simulink model "ElectricVehicleThermalManagementWithHeatPump"  (R2024b)
settings: Solver=VariableStepAuto  StartTime=0.0  StopTime=3600  RelTol=1e-3  AbsTol=1e-3
PreLoadFcn:
  | init_nmpc
InitFcn:
  | init_nmpc
model workspace: external: MATLAB File ElectricVehicleThermalManagementWithHeatPumpParameters.m (data not in the file)
values from neighbouring files (symbols this model uses):
  battery_C1_LUT = [1913.6 12447 30609 ... (first row only)    [ElectricVehicleThermalManagementWithHeatPumpParameters.m]
  battery_capacity_LUT = [280.081 276.25 276.392]    [ElectricVehicleThermalManagementWithHeatPumpParameters.m]
  battery_cell_cp = 795    [ElectricVehicleThermalManagementWithHeatPumpParameters.m]
  battery_cell_mass = 2.5    [ElectricVehicleThermalManagementWithHeatPumpParameters.m]
  battery_Em_LUT = [3.4966 3.5057 3.5148 ... (first row only)    [ElectricVehicleThermalManagementWithHeatPumpParameters.m]
  battery_N_cells = 20    [ElectricVehicleThermalManagementWithHeatPumpParameters.m]
  battery_Qe_init = 0    [ElectricVehicleThermalManagementWithHeatPumpParameters.m]
  battery_R0_LUT = [0.0117 0.0085 0.009 ... (first row only)    [ElectricVehicleThermalManagementWithHeatPumpParameters.m]
  battery_R1_LUT = [0.0109 0.0029 0.0013 ... (first row only)    [ElectricVehicleThermalManagementWithHeatPumpParameters.m]
  battery_SOC_LUT = [0; 0.1; 0.25; 0.5; 0.75; 0.9; 1]    [ElectricVehicleThermalManagementWithHeatPumpParameters.m]
  battery_T_init = -10    [ElectricVehicleThermalManagementWithHeatPumpParameters.m]
  battery_temperature_LUT = [5 20 40]    [ElectricVehicleThermalManagementWithHeatPumpParameters.m]
  cabin_duct_area = 0.04    [ElectricVehicleThermalManagementWithHeatPumpParameters.m]
  cabin_T_init = -10    [ElectricVehicleThermalManagementWithHeatPumpParameters.m]
  chiller_area_primary = 0.43982297150257105    (= 0.439822971503)    [ElectricVehicleThermalManagementWithHeatPumpParameters.m]
  chiller_N_baffles = 3    [ElectricVehicleThermalManagementWithHeatPumpParameters.m]
  chiller_N_tubes = 100    [ElectricVehicleThermalManagementWithHeatPumpParameters.m]
  chiller_tube_D = 0.0035    [ElectricVehicleThermalManagementWithHeatPumpParameters.m]
  chiller_tube_L = 0.4    [ElectricVehicleThermalManagementWithHeatPumpParameters.m]
  chiller_wall_conductivity = 240    [ElectricVehicleThermalManagementWithHeatPumpParameters.m]
  chiller_wall_thickness = 0.0001    [ElectricVehicleThermalManagementWithHeatPumpParameters.m]
  cond_evap_air_area_flow = 0.3906    [ElectricVehicleThermalManagementWithHeatPumpParameters.m]
  cond_evap_air_area_primary = 1.4834999999999998    (= 1.4835)    [ElectricVehicleThermalManagementWithHeatPumpParameters.m]
  cond_evap_W = 0.015    [ElectricVehicleThermalManagementWithHeatPumpParameters.m]
  cond_evap_wall_conductivity = 240    [ElectricVehicleThermalManagementWithHeatPumpParameters.m]
  cond_evap_wall_thickness = 0.0001    [ElectricVehicleThermalManagementWithHeatPumpParameters.m]
  coolant_channel_D = 0.0092    [ElectricVehicleThermalManagementWithHeatPumpParameters.m]
  coolant_pipe_D = 0.019    [ElectricVehicleThermalManagementWithHeatPumpParameters.m]
  coolant_T_init = -10    [ElectricVehicleThermalManagementWithHeatPumpParameters.m]
  coolant_tank_area = 0.0121    [ElectricVehicleThermalManagementWithHeatPumpParameters.m]
  coolant_tank_volume = 1.25    [ElectricVehicleThermalManagementWithHeatPumpParameters.m]
  coolant_valve_D_ratio_max = 0.95    [ElectricVehicleThermalManagementWithHeatPumpParameters.m]
  coolant_valve_D_ratio_min = 0.001    [ElectricVehicleThermalManagementWithHeatPumpParameters.m]
  coolant_valve_displacement = 0.0063    [ElectricVehicleThermalManagementWithHeatPumpParameters.m]
  coolant_valve_S_max = 0.0053    [ElectricVehicleThermalManagementWithHeatPumpParameters.m]
  evaporator_air_area_flow = 0.12    [ElectricVehicleThermalManagementWithHeatPumpParameters.m]
  evaporator_air_area_primary = 0.4323    [ElectricVehicleThermalManagementWithHeatPumpParameters.m]
  evaporator_W = 0.015    [ElectricVehicleThermalManagementWithHeatPumpParameters.m]
  evaporator_wall_conductivity = 240    [ElectricVehicleThermalManagementWithHeatPumpParameters.m]
  evaporator_wall_thickness = 0.0001    [ElectricVehicleThermalManagementWithHeatPumpParameters.m]
  expansion_valve_D_ratio_max = 0.9    [ElectricVehicleThermalManagementWithHeatPumpParameters.m]
  hex_area_primary = 0.070371675440411369    (= 0.0703716754404)    [ElectricVehicleThermalManagementWithHeatPumpParameters.m]
  hex_N_tubes = 64    [ElectricVehicleThermalManagementWithHeatPumpParameters.m]
  hex_tube_D = 0.0035    [ElectricVehicleThermalManagementWithHeatPumpParameters.m]
  hex_wall_conductivity = 240    [ElectricVehicleThermalManagementWithHeatPumpParameters.m]
  hex_wall_thickness = 0.0001    [ElectricVehicleThermalManagementWithHeatPumpParameters.m]
  inner_cond_air_area_flow = 0.1953    [ElectricVehicleThermalManagementWithHeatPumpParameters.m]
  inner_cond_air_area_primary = 0.99520000000000008    (= 0.9952)    [ElectricVehicleThermalManagementWithHeatPumpParameters.m]
  inner_cond_W = 0.02    [ElectricVehicleThermalManagementWithHeatPumpParameters.m]
  inner_cond_wall_conductivity = 240    [ElectricVehicleThermalManagementWithHeatPumpParameters.m]
  inner_cond_wall_thickness = 0.0001    [ElectricVehicleThermalManagementWithHeatPumpParameters.m]
  pump_speed_max = 1000    [ElectricVehicleThermalManagementWithHeatPumpParameters.m]
  radiator_air_area_flow = 0.097499999999999989    (= 0.0975)    [ElectricVehicleThermalManagementWithHeatPumpParameters.m]
  radiator_air_area_primary = 0.43687499999999996    (= 0.436875)    [ElectricVehicleThermalManagementWithHeatPumpParameters.m]
  radiator_W = 0.015    [ElectricVehicleThermalManagementWithHeatPumpParameters.m]
  radiator_wall_conductivity = 240    [ElectricVehicleThermalManagementWithHeatPumpParameters.m]
  radiator_wall_thickness = 0.0001    [ElectricVehicleThermalManagementWithHeatPumpParameters.m]
  refrigerant_p_init = 0.2    [ElectricVehicleThermalManagementWithHeatPumpParameters.m]
  refrigerant_pipe_D = 0.01    [ElectricVehicleThermalManagementWithHeatPumpParameters.m]
  refrigerant_valve_D_ratio_max = 0.95    [ElectricVehicleThermalManagementWithHeatPumpParameters.m]
  refrigerant_valve_displacement = 0.005    [ElectricVehicleThermalManagementWithHeatPumpParameters.m]
libraries: fl_lib x227, nesl_utility x162, SimscapeFluids_lib x30, LiBatteryElements_lib x16, slpidlib x3, SignalEditorBlockLib x1
(part 2 of 13)

== system ElectricVehicleThermalManagementWithHeatPump/Battery Pump ==
  Battery Coolant Tank : SimscapeFluids_lib/Thermal Liquid/Tanks & Accumulators/Tank (G-TL)  num_inlet=2  volume_total=coolant_tank_volume l  volume_spec=1  tank_area=coolant_tank_area m^2  level_TLU=[0, 3, 5] m  volume_TLU=[0, 4, 6] m^3  inlet_areas_A1B1=[.01, .01] m^2  inlet_height_A2=0.1 m  inlet_area_A2=0.01 m^2  inlet_heights_A2B2=[0, 0] m  inlet_areas_A2B2=[1 1] * pi * coolant_pipe_D^2 / 4 m^2  inlet_heights_A2B2C2=[.1, .05, 0] m  inlet_areas_A2B2C2=[.01, .01, .01] m^2  inlet_heights_A2B2C2D2=0.1 * ones(1, 4) m  inlet_areas_A2B2C2D2=0.01 * ones(1, 4) m^2  inlet_heights_A2B2C2D2E2=0.1 * ones(1, 5) m  inlet_areas_A2B2C2D2E2=0.01 * ones(1, 5) m^2  inlet_heights_A2B2C2D2E2F2=0.1 * ones(1, 6) m  inlet_areas_A2B2C2D2E2F2=0.01 * ones(1, 6) m^2  capacity_check=0  max_liquid_capacity=coolant_tank_volume l  g=0 m/s^2  level_specify=on  level_priority=None  level=5 m  level_nominal_specify=off  level_nominal_value=1  level_nominal_unit=m  volume_liquid_specify=on  volume_liquid_priority=High  volume_liquid=0.25 * coolant_tank_volume l  volume_liquid_nominal_specify=off  volume_liquid_nominal_value=1  volume_liquid_nominal_unit=m^3  mass_liquid_specify=off  mass_liquid_priority=None  mass_liquid=5e+3 kg  mass_liquid_nominal_specify=off  mass_liquid_nominal_value=1  mass_liquid_nominal_unit=kg  T_liquid_specify=on  T_liquid_priority=High  T_liquid=coolant_T_init degC  T_liquid_nominal_specify=off  T_liquid_nominal_value=1  T_liquid_nominal_unit=K  p_gas_specify=on  p_gas_priority=High  p_gas=coolant_p_init MPa  p_gas_nominal_specify=off  p_gas_nominal_value=1  p_gas_nominal_unit=MPa  T_gas_specify=on  T_gas_priority=High  T_gas=coolant_T_init degC  T_gas_nominal_specify=off  T_gas_nominal_value=1  T_gas_nominal_unit=K  rho_gas_specify=off  rho_gas_priority=None  rho_gas=1.2 kg/m^3  rho_gas_nominal_specify=off  rho_gas_nominal_value=1  rho_gas_nominal_unit=kg/m^3
      settings: InternalSimscapePortConfiguration="{\"Bottom\":[],\"Left\":[{\"id\":\"A1\",\"label\":\"A1\",\"type\":\"foundation.gas.gas\"},{\"id\":\"B1\",\"label\":\"B1\",\"type\":\"foundation.gas.gas\"},{\"id\":\"A2\",\"label\":\"A2\",\"type\":\"foundation.thermal_liquid.thermal_liquid\"},{\"id\":\"B2\",\"label\":\"B2\",\"type\":\"foundation.thermal_liquid.thermal_liquid\"}],\"Right\":[{\"id\":\"H1\",\"label\":\"H1\",\"type\":\"foundation.thermal.thermal\"},{\"id\":\"H2\",\"label\":\"H2\",\"type\":\"foundation.thermal.thermal\"}],\"Top\":[{\"id\":\"V_out\",\"label\":\"V\",\"type\":\"output\"},{\"id\":\"L_out\",\"label\":\"L\",\"type\":\"output\"}]}"
  Battery Pump : SimscapeFluids_lib/Thermal Liquid/Pumps & Motors/Fixed-Displacement Pump (TL)  loss_spec=1  displacement=pump_displacement l/rev  omega_nominal=0.5 * pump_speed_max rpm  p_nominal=0.1 MPa  mu_nominal=0.9 cP  vol_eff_nominal=0.92  mech_eff_nominal=0.88  no_load_torque=0.03 N*m  p_diff_eff_TLU=[.1, 1, 2] MPa  omega_eff_TLU=[25, 50, 100, 200, 300, 400] rad/s  vol_eff_TLU=[.816, .908, .954, .977, .981, .984; .325, .663, .831, .916, .925, .946; .137, .568, .78, .892, .893, .91]  mech_eff_TLU=[.996, .996, .996, .996, .996, .996; .988, .989, .989, .989, .989, .99; .981, .981, .982, .982, .983, .984]  p_diff_loss_TLU=[.1, 1, 2] MPa  omega_loss_TLU=[25, 50, 100, 200, 300, 400] rad/s  vol_loss_TLU=[.023, .023, .023, .023, .0285, .032; .0844, .0842, .0845, .084, .1125, .108; .1079, .108, .11, .108, .1605, .18] * 1e-3 m^3/s  mech_loss_TLU=[.002, .002, .002, .002, .002, .002; .0607, .0556, .0556, .0556, .0556, .0505; .1937, .1937, .1833, .1833, .1729, .1626] N*m  vol_eff_min=1e-3  vol_eff_max=1  mech_eff_min=1e-3  mech_eff_max=1  pressure_threshold=1e-3 MPa  omega_threshold=10 rad/s  area=pi * coolant_pipe_D^2 / 4 m^2  supplied_range_check=0  pump_mode_check=simscape.enum.assert.action.none  pressure_check=simscape.enum.assert.action.none  p_min_valid=0.101325 MPa
  Cap (G) : fl_lib/Gas/Elements/Cap (G)  p_specify=off  p_priority=None  p=0.101325 MPa  p_nominal_specify=off  p_nominal_value=1  p_nominal_unit=MPa  T_specify=off  T_priority=None  T=293.15 K  T_nominal_specify=off  T_nominal_value=1  T_nominal_unit=K
  Cap (G)1 : fl_lib/Gas/Elements/Cap (G)  p_specify=off  p_priority=None  p=0.101325 MPa  p_nominal_specify=off  p_nominal_value=1  p_nominal_unit=MPa  T_specify=off  T_priority=None  T=293.15 K  T_nominal_specify=off  T_nominal_value=1  T_nominal_unit=K
  Flow Rate Sensor (TL) : fl_lib/Thermal Liquid/Sensors/Flow Rate Sensor (TL)  mass_flow_measure=true  volumetric_flow_measure=false  energy_flow_measure=true
      settings: InternalSimscapePortConfiguration="{\"Bottom\":[{\"id\":\"PHI\",\"label\":\"φ\",\"type\":\"output\"}],\"Left\":[{\"id\":\"A\",\"label\":\"A\",\"type\":\"foundation.thermal_liquid.thermal_liquid\"}],\"Right\":[{\"id\":\"B\",\"label\":\"B\",\"type\":\"foundation.thermal_liquid.thermal_liquid\"},{\"id\":\"M\",\"label\":\"M\",\"type\":\"output\"}],\"Top\":[]}"
  Flow Rate Sensor (TL)1 : fl_lib/Thermal Liquid/Sensors/Flow Rate Sensor (TL)  mass_flow_measure=true  volumetric_flow_measure=false  energy_flow_measure=true
      settings: InternalSimscapePortConfiguration="{\"Bottom\":[{\"id\":\"PHI\",\"label\":\"φ\",\"type\":\"output\"}],\"Left\":[{\"id\":\"A\",\"label\":\"A\",\"type\":\"foundation.thermal_liquid.thermal_liquid\"}],\"Right\":[{\"id\":\"B\",\"label\":\"B\",\"type\":\"foundation.thermal_liquid.thermal_liquid\"},{\"id\":\"M\",\"label\":\"M\",\"type\":\"output\"}],\"Top\":[]}"
  Heat Transfer : Subsystem
  Ideal Angular Velocity Source : fl_lib/Mechanical/Mechanical Sources/Ideal Angular Velocity Source
  Max Speed [rpm] : Gain  Gain=4000
  Mechanical Rotational Reference : fl_lib/Mechanical/Rotational Elements/Mechanical Rotational Reference
  PS-Simulink Converter : nesl_utility/PS-Simulink Converter  PhysicalDomain=network_engine_domain  SubClassName=ps_output  LeftPortType=input  RightPortType=output  PseudoPeriodic=off  Frequencies=[]  VectorFormat=inherit  Unit=kg/s  AffineConversion=off
  PS-Simulink Converter1 : nesl_utility/PS-Simulink Converter  PhysicalDomain=network_engine_domain  SubClassName=ps_output  LeftPortType=input  RightPortType=output  PseudoPeriodic=off  Frequencies=[]  VectorFormat=inherit  Unit=inherit  AffineConversion=off
  Scope : Scope
  Scope1 : Scope
  Simulink-PS Converter : nesl_utility/Simulink-PS Converter  PhysicalDomain=network_engine_domain  SubClassName=ps_input  LeftPortType=input  RightPortType=output  PseudoPeriodic=off  Frequencies=[]  NoiseDistribution=none  NoiseParameters=[]  Unit=rpm  AffineConversion=off  FilteringAndDerivatives=provide  SimscapeFilterOrder=1  InputFilterTimeConstant=0.001  UdotUserProvided=0
  Switch : Switch  Criteria=u2 > Threshold  SaturateOnIntegerOverflow=off  InputSameDT=off
  Transfer Fcn : TransferFcn  Denominator=[5 1]
  Transfer Fcn1 : TransferFcn  Denominator=[5 1]
  A : PMIOPort  Side=Left
  B : PMIOPort  Port=2  Side=Right
  wires:
  Transfer Fcn/1 -> Max Speed [rpm]/1
  [cmd_battery_pump] -> Transfer Fcn/1
  PS-Simulink Converter/1 -> Scope/1
  PS-Simulink Converter1/1 -> Scope1/1
  [batPumpNrpm] -> Transfer Fcn1/1
  [MPCController] -> Switch/2
  Max Speed [rpm]/1 -> Switch/3
  Switch/1 -> Simulink-PS Converter/1
  Transfer Fcn1/1 -> Switch/1
  connections:
  Mechanical Rotational Reference/LConn1 -- Ideal Angular Velocity Source/RConn2 -- Battery Pump/RConn2
  Simulink-PS Converter/RConn1 -- Ideal Angular Velocity Source/RConn1
  Ideal Angular Velocity Source/LConn1 -- Battery Pump/RConn1
  A/RConn1 -- Battery Coolant Tank/LConn3 -- Flow Rate Sensor (TL)/LConn1
  Cap (G)1/LConn1 -- Battery Coolant Tank/LConn2
  Heat Transfer/RConn2 -- Battery Coolant Tank/RConn2
  Cap (G)/LConn1 -- Battery Coolant Tank/LConn1
  Battery Pump/LConn1 -- Battery Coolant Tank/LConn4
  Heat Transfer/RConn1 -- Battery Coolant Tank/RConn1
  Flow Rate Sensor (TL)/RConn2 -- PS-Simulink Converter/LConn1
  Flow Rate Sensor (TL)1/RConn1 -- Battery Pump/LConn2
  Flow Rate Sensor (TL)1/LConn1 -- B/RConn1
  PS-Simulink Converter1/LConn1 -- Flow Rate Sensor (TL)1/RConn2

== system ElectricVehicleThermalManagementWithHeatPump/Blend Door ==
  Blend Door : Subsystem  Tag=PublishSubsystem  mask{min_area=1e-8 * cabin_duct_area, max_area=0.9 * cabin_duct_area, port_area=cabin_duct_area, Cd=0.8, tau=1}
      mask prompts: min_area "Min restriction area (m^2)"; max_area "Max restriction area (m^2)"; port_area "Cross-sectional area at ports A, B, and C (m^2)"; Cd "Discharge coefficient"; tau "Opening time constant (s)"
      settings: PortSchema="{\"entries\":[{\"content\":{\"sides\":[{\"content\":{\"connectorIds\":[\"LConn1\"]},\"type\":\"ConnectorPlacement.EquallySpacedRectSide\",\"uuid\":\"701091b4-901c-43e1-a8a1-50bf4fd327d1\"},{\"content\":{\"connectorIds\":[\"RConn1\"],\"side\":\"RIGHT\"},\"type\":\"ConnectorPlacement.EquallySpacedRectSide\",\"uuid\":\"6ee33cdd-bbd1-4683-8a8c-22edb39550e2\"},{\"content\":{\"side\":\"TOP\"},\"type\":\"ConnectorPlacement.EquallySpacedRectSide\",\"uuid\":\"c0b8be11-b43c-4098-95a0-d44066221ea6\"},{\"content\":{\"connectorIds\":[\"RConn2\"],\"side\":\"BOTTOM\"},\"type\":\"ConnectorPlacement.EquallySpacedRectSide\",\"uuid\":\"1c585638-1e64-4636-940b-c407bc21f999\"}]},\"type\":\"ConnectorPlacement.EquallySpacedConnector\",\"uuid\":\"9280612b-569a-4615-9ade-e87314c5223e\"}],\"packageUris\":[\"http://schema.mathworks.com/mf0/Connector/R2020b\"],\"version\":\"1.0\"}"
  A : PMIOPort  Side=Left
  B : PMIOPort  Port=2  Side=Right
  C : PMIOPort  Port=3  Side=Right
  connections:
  Blend Door/LConn1 -- A/RConn1
  B/RConn1 -- Blend Door/RConn1
  C/RConn1 -- Blend Door/RConn2

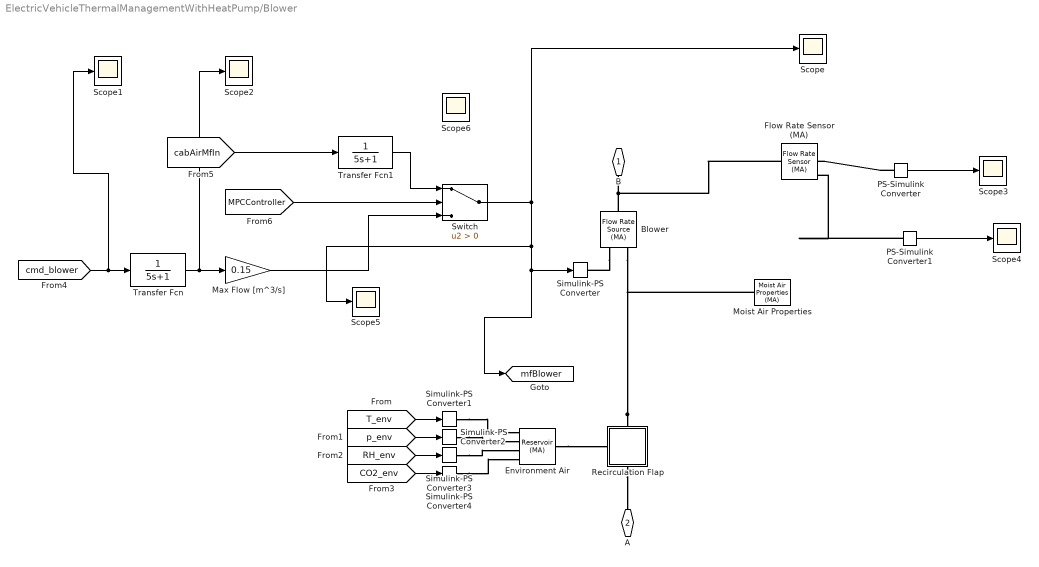
== system ElectricVehicleThermalManagementWithHeatPump/Blower ==
  Blower : fl_lib/Moist Air/Sources/Flow Rate Source (MA)  source_type=foundation.enum.constant_controlled.controlled  flow_type=foundation.enum.mass_volumetric_flow.volumetric  mass_flow=0 kg/s  volumetric_flow=0 m^3/s  volumetric_flow_conditions=foundation.enum.volumetric_flow_conditions.actual  p_std=0.101325 MPa  T_std=20 degC  RH_std=0.65  power_spec=foundation.enum.power_spec.isentropic  area_A=cabin_duct_area m^2  area_B=cabin_duct_area m^2
      settings: InternalSimscapePortConfiguration="{\"Bottom\":[],\"Left\":[{\"id\":\"A\",\"label\":\"A\",\"type\":\"foundation.moist_air.moist_air\"},{\"id\":\"V\",\"label\":\"V\",\"type\":\"input\"}],\"Right\":[{\"id\":\"B\",\"label\":\"B\",\"type\":\"foundation.moist_air.moist_air\"}],\"Top\":[]}"
  Environment Air : fl_lib/Moist Air/Elements/Reservoir (MA)  pressure_input=true  pressure_spec=foundation.enum.pressure_spec.atmospheric  reservoir_pressure=0.101325 MPa  temperature_input=true  temperature_spec=foundation.enum.temperature_spec.atmospheric  reservoir_temperature=293.15 K  humidity_input=true  humidity_spec=foundation.enum.HumiditySpec.RelativeHumidity  reservoir_RH=0.5  reservoir_x_w=0.01  reservoir_y_w=0.01  reservoir_HR=0.01  reservoir_Tw=287 K  trace_gas_input=true  trace_gas_spec=foundation.enum.trace_gas_spec.mole_fraction  reservoir_x_g=0.001  reservoir_y_g=0.001  water_droplets_input=false  reservoir_r_d=0  RH_ws=1  area_A=cabin_duct_area m^2  input_error_spec=foundation.enum.input_range_error.warn
      settings: InternalSimscapePortConfiguration="{\"Bottom\":[],\"Left\":[{\"id\":\"A\",\"label\":\"A\",\"type\":\"foundation.moist_air.moist_air\"}],\"Right\":[{\"id\":\"T\",\"label\":\"T\",\"type\":\"input\"},{\"id\":\"P\",\"label\":\"P\",\"type\":\"input\"},{\"id\":\"W\",\"label\":\"W\",\"type\":\"input\"},{\"id\":\"G\",\"label\":\"G\",\"type\":\"input\"}],\"Top\":[]}"
  Flow Rate Sensor (MA) : fl_lib/Moist Air/Sensors/Flow Rate Sensor (MA)  mass_flow_measure=true  volumetric_flow_measure=false  volumetric_flow_conditions=foundation.enum.volumetric_flow_conditions.actual  p_std=0.101325 MPa  T_std=20 degC  RH_std=0.65  energy_flow_measure=true  vapor_flow_measure=false  gas_flow_measure=false  droplets_flow_measure=false
      settings: InternalSimscapePortConfiguration="{\"Bottom\":[{\"id\":\"PHI\",\"label\":\"φ\",\"type\":\"output\"}],\"Left\":[{\"id\":\"A\",\"label\":\"A\",\"type\":\"foundation.moist_air.moist_air\"}],\"Right\":[{\"id\":\"B\",\"label\":\"B\",\"type\":\"foundation.moist_air.moist_air\"},{\"id\":\"M\",\"label\":\"M\",\"type\":\"output\"}],\"Top\":[]}"
  Max Flow [m^3/s] : Gain  Gain=0.15
  Moist Air Properties : fl_lib/Moist Air/Utilities/Moist Air Properties (MA)  R_a=287.047 J/(K*kg)  T_TLU=[-56.55, -50 : 10 : -10, -5 : 1 : 5, 10 : 10 : 350]' degC  h_a_TLU=[342.414066793634; 349.003411914139; 359.061417476782; 369.117728274935; 379.173188407993; 389.228602960013; 394.256538873206; 395.262156814682; 396.26778682262; 397.27342967397; 398.279086145689; 399.284757014822; 400.290443058569; 401.296145054364; 402.301863779931; 403.307600013352; 404.313354533128; 409.342428711098; 419.402397945314; 429.465451846544; 439.532387826623; 449.604014793745; 459.68115297076; 469.764632657687; 479.855292205971; 489.953975419749; 500.06152856014; 510.178797098051; 520.306622336267; 530.445838000969; 540.597266885076; 550.761717610289; 560.939981561004; 571.132830031086; 581.341011613777; 591.565249855533; 601.806241186423; 612.064653132654; 622.341122810862; 632.636255698901; 642.95062467384; 653.284769304793; 663.639195385783; 674.014374692179; 684.410744943084; 694.828709951456; 705.268639943519; 715.730872029167; 726.215710805484; 736.723429076127; 747.254268670154; 757.808441344776] kJ/kg  mu_a_TLU=[14.2568884161326; 14.6140128551699; 15.151727785151; 15.6806860927178; 16.201235181264; 16.7137043838401; 16.9670072430524; 17.017438132541; 17.0677931537044; 17.1180726001803; 17.1682767640582; 17.2184059358881; 17.2684604046898; 17.318440457962; 17.3683463816913; 17.4181784603614; 17.467936976962; 17.7156359301048; 18.2056752419787; 18.6887904184394; 19.1652345249932; 19.6352479488881; 20.099059157425; 20.5568854116507; 21.008933436444; 21.4554000485251; 21.8964727442509; 22.3323302492491; 22.7631430320408; 23.1890737838183; 23.6102778665211; 24.0269037312887; 24.4390933092858; 24.8469823767971; 25.2507008963847; 25.6503733357905; 26.0461189661617; 26.438052141067; 26.8262825576728; 27.210915501349; 27.5920520748824; 27.969789413389; 28.3442208859359; 28.7154362848061; 29.0835220032714; 29.4485612026716; 29.8106339695395; 30.169817463453; 30.5261860562487; 30.8798114631771; 31.2307628665438; 31.5791070323335] s*uPa  k_a_TLU=[19.8808491891482; 20.4162457047568; 21.2248745869044; 22.0232455041378; 22.8117316528767; 23.59069155438; 23.9767077285082; 24.0536401764626; 24.130482853517; 24.2072360894785; 24.2839002127411; 24.3604755502875; 24.4369624276914; 24.5133611691197; 24.5896720973349; 24.6658955336975; 24.7420317981691; 25.1214166432482; 25.8738284673185; 26.6180151791963; 27.3542675863918; 28.0828636150405; 28.8040688184917; 29.5181369069754; 30.2253102842368; 30.9258205811167; 31.6198891790667; 32.307727718801; 32.989538590917; 33.6655154065126; 34.3358434467079; 35.0007000906151; 35.6602552217624; 36.314671613305; 36.9641052925838; 37.6087058857479; 38.2486169432557; 38.8839762471259; 39.5149161008418; 40.1415636028127; 40.7640409042923; 41.3824654526272; 41.9969502206863; 42.6076039232795; 43.2145312213471; 43.8178329146528; 44.4176061236819; 45.0139444614019; 45.6069381955058; 46.1966744017242; 46.7832371087507; 47.3667074352967] mW/(K*m)  p_min=1 kPa  p_max=inf MPa  T_min=-56.55 degC  T_max=350 degC  properties_range_check=simscape.enum.assert.action.error  p_atm=0.101325 MPa  T_atm=20 degC  enable_droplets=false  R_w=461.523 J/(K*kg)  p_ws_TLU=[1.71168953425982e-06; 3.93770601979424e-06; 1.28411717710344e-05; 3.80051394873809e-05; .00010323902900209; .000259873810798063; .000401741022116384; .000437454836117844; .000476040820618202; .000517704666185737; .000562664883741207; .000611212677444345; .000657085634113763; .000705985593917791; .00075808051438111; .000813548355379396; .000872575113841924; .00122819910164487; .00233931836947519; .00424697076171126; .00738493802968097; .012351945812707; .0199464343236764; .0312009300307261; .0474144740241604; .0701817658485933; .101417996663294; .143378712947169; .198674420476403; .270279976781692; .361539099388177; .476164537971214; .618234621423587; .792187006980199; 1.00281053608169; 1.25523615516845; 1.55492790046272; 1.90767499353199; 2.31958617020155; 2.79708749692822; 3.34692514426746; 3.97617493064794; 4.69226099229504; 5.50298678300951; 6.41658290952841; 7.44177834442093; 8.58790494083256; 9.86505121117553; 11.284292927457; 12.8580516000122; 14.6006773719404; 16.5294151389953] MPa  h_w_vap_TLU=[2836.88241275372; 2837.81392500514; 2838.63937175807; 2838.7309929628; 2838.06905313927; 2836.62597341095; 2835.60023952573; 2835.37006381376; 2835.13143158077; 2834.88429145066; 2834.62859062897; 2500.93420564316; 2498.55452890293; 2496.17317793437; 2493.7941260618; 2491.41713708944; 2489.04199020767; 2477.18706302224; 2453.51925941961; 2429.81122987564; 2405.97728678685; 2381.94712654051; 2357.65452030374; 2333.03120800924; 2308.00352809267; 2282.49062771796; 2256.40372152657; 2229.64615315163; 2202.11407337172; 2173.6974807639; 2144.28128268553; 2113.74600964951; 2081.9678834089; 2048.81807129851; 2014.16109962579; 1977.85249331179; 1939.73572816654; 1899.63852389863; 1857.36838273035; 1812.70710332357; 1765.4037880462; 1715.16561416478; 1661.64526339623; 1604.4232249434; 1542.98206457018; 1476.66790089115; 1404.63083498414; 1325.72875296442; 1238.36212284382; 1140.16281350074; 1027.31658328826; 892.746804215825] kJ/kg  h_w_TLU=[2396.53078650168; 2408.65722023252; 2427.16766028467; 2445.66624034104; 2464.1379798878; 2482.5594701893; 2491.7412703989; 2493.57467660537; 2495.40699233755; 2497.23816944599; 2499.06815833272; 2500.89261781717; 2502.73123919979; 2504.56496564907; 2506.39800457704; 2508.23033644628; 2510.06194120626; 2519.20831890725; 2537.43340437276; 2555.54520329515; 2573.51032237465; 2591.28888786817; 2608.83487221908; 2626.09640083333; 2643.01588134754; 2659.53001419864; 2675.5827869577; 2696.18462565746; 2716.49989554204; 2736.6235211014; 2756.61216047677; 2776.50561774616; 2796.33378923373; 2816.11979584021; 2835.88181424959; 2855.6343057571; 2875.38889328914; 2895.15500578618; 2914.94035966265; 2934.75132291939; 2954.59319332093; 2974.47041287496; 2994.38673461102; 3014.34535330297; 3034.34900869544; 3054.40006758361; 3074.50058949656; 3094.65237956705; 3114.85703131193; 3135.11596141057; 3155.43043809331; 3175.80160439414] kJ/kg  mu_w_TLU=[6.9886414857741; 7.21462000349698; 7.55962537406626; 7.90463074463554; 8.24963611520482; 8.5946414857741; 8.76714417105874; 8.80164470811567; 8.8361452451726; 8.87064578222952; 8.90514631928645; 8.93964685634338; 8.97414739340031; 9.00294911497154; 9.0318980288863; 9.06099135942002; 9.09022638806001; 9.23843559844524; 9.5440595677542; 9.86015858692705; 10.1848429274122; 10.5164578096049; 10.8535319382781; 11.1947482575333; 11.5389294976352; 11.8850331780701; 12.2322493177351; 12.6188533568459; 13.0082793358938; 13.4003380262893; 13.7948421428098; 14.1916095618232; 14.590464747099; 14.9912394314964; 15.3937729006119; 15.7979120385447; 16.203511226482; 16.610432150303; 17.0185435533718; 17.4277209582061; 17.8378463726577; 18.2488079909412; 18.6604998963166; 19.0728217698535; 19.485678608085; 19.8989804512625; 20.3126421231677; 20.7265829829225; 21.1407266888906; 21.5550009745266; 21.969337435876; 22.3836713303269] s*uPa  k_w_TLU=[12.4916816538045; 12.9847788176262; 13.737598915064; 14.4904190125018; 15.2432391099396; 15.9960592073774; 16.3724692560963; 16.4477512658401; 16.5230332755839; 16.5983152853277; 16.6735972950715; 16.7488793048152; 16.824161314559; 16.8886088206517; 16.9532779906513; 17.0181691764255; 17.083282769915; 17.4122036181723; 18.0870861656185; 18.7855813517187; 19.5093466408385; 20.2607864040347; 21.0430876297671; 21.8602068151121; 22.7168164077153; 23.6182141540994; 24.5698636875305; 25.4024944426483; 26.2458938647479; 27.1009155051916; 27.968142896353; 28.8479507975112; 29.7405485790829; 30.646029672269; 31.5643932662527; 32.4955693285114; 33.4394360046859; 34.3958329885356; 35.3645718140131; 36.3454437886179; 37.3382261129791; 38.3426866012072; 39.3585873185985; 40.3856873794121; 41.4237450915028; 42.4725195920623; 43.5317720862424; 44.6012667755489; 45.6807715437344; 46.7700584531355; 47.8689040929333; 48.9770898119082] mW/(K*m)  D_w=25 mm^2/s  trace_gas_model=foundation.enum.trace_gas_model.track_fraction  R_g=188.923 J/(K*kg)  h_g_TLU=[439.555216276024; 444.670268214299; 452.538618857965; 460.487124266174; 468.522588773143; 476.64941595933; 480.747985385885; 481.570543185868; 482.394052396612; 483.218514286302; 484.043930026094; 484.87030069324; 485.697627274149; 486.525910667382; 487.355151686572; 488.185351063277; 489.016509449741; 493.186704132078; 501.599194941473; 510.107689945701; 518.711611059603; 527.410026767716; 536.20176474847; 545.085474167968; 554.059675464379; 563.122805439004; 572.273250917104; 581.509372969931; 590.829525041787; 600.232066635428; 609.715373504524; 619.277845094572; 628.91790983254; 638.634028741375; 648.424697754692; 658.288449028076; 668.22385148184; 678.229510761734; 688.30406876583; 698.446202855373; 708.654624842952; 718.928079831753; 729.265344963773; 739.665228122078; 750.126566621791; 760.648225916092; 771.229098336723; 781.86810188302; 792.564179069104; 803.316295835373; 814.123440527678; 824.984622945405] kJ/kg  mu_g_TLU=[10.9386626034033; 11.2618160869372; 11.7542862475187; 12.2454955799777; 12.7352208796158; 13.2232325321233; 13.4665248390743; 13.5151226761166; 13.5636997995993; 13.6122559954699; 13.6607910510226; 13.709304754931; 13.757796897279; 13.8062672695897; 13.8547156648526; 13.9031418775498; 13.9515457036801; 14.1932220047332; 14.6747828595747; 15.153802214283; 15.6301123398299; 16.1035631756244; 16.574022106427; 17.0413733976215; 17.5055174102327; 17.9663696812767; 18.4238599299346; 18.8779310322956; 19.3285379947687; 19.7756469471288; 20.2192341695255; 20.6592851629269; 21.0957937689132; 21.5287613421341; 21.9581959768344; 22.3841117874779; 22.8065282425078; 23.2254695495877; 23.6409640901974; 24.0530439011453; 24.4617442003854; 24.8671029544344; 25.269160484669; 25.6679591098169; 26.0635428220247; 26.4559569939835; 26.8452481147025; 27.2314635516519; 27.6146513371198; 27.9948599767665; 28.3721382784874; 28.74653519983] s*uPa  k_g_TLU=[10.7373095949238; 11.1772934980884; 11.862915506018; 12.5638333280734; 13.2785475592421; 14.005722199619; 14.3736017704762; 14.4475028211958; 14.5215096973787; 14.5956213250986; 14.6698366403414; 14.7441545888563; 14.8185741260114; 14.8930942166532; 14.9677138349692; 15.0424319643548; 15.1172475972825; 15.4927536712633; 16.2505237772467; 17.0165521650722; 17.7899991951805; 18.5700903932503; 19.3561099002839; 20.1473949639617; 20.9433312278214; 21.7433486448307; 22.5469178892132; 23.3535471729555; 24.1627793965491; 24.9741895799701; 25.7873825314493; 26.6019907190427; 27.4176723115859; 28.2341093347412; 29.0510055857402; 29.8680879651392; 30.6851034165693; 31.5018116707882; 32.3179924018673; 33.1334410491403; 33.9479677779769; 34.7613965127281; 35.5735640361829; 36.3843191504339; 37.1935218945334; 38.0010428147395; 38.80676228352; 39.6105698638057; 40.412363715274; 41.2120500397018; 42.0095425626597; 42.8047620490288] mW/(K*m)  D_g=16 mm^2/s
  PS-Simulink Converter : nesl_utility/PS-Simulink Converter  PhysicalDomain=network_engine_domain  SubClassName=ps_output  LeftPortType=input  RightPortType=output  PseudoPeriodic=off  Frequencies=[]  VectorFormat=inherit  Unit=inherit  AffineConversion=off
  PS-Simulink Converter1 : nesl_utility/PS-Simulink Converter  PhysicalDomain=network_engine_domain  SubClassName=ps_output  LeftPortType=input  RightPortType=output  PseudoPeriodic=off  Frequencies=[]  VectorFormat=inherit  Unit=inherit  AffineConversion=off
  Recirculation Flap : Subsystem  Tag=PublishSubsystem  mask{min_area=1e-8 * cabin_duct_area, max_area=0.9 * cabin_duct_area, port_area=cabin_duct_area, Cd=0.8, tau=1}
      mask prompts: min_area "Min restriction area (m^2)"; max_area "Max restriction area (m^2)"; port_area "Cross-sectional area at ports A, B, and C (m^2)"; Cd "Discharge coefficient"; tau "Opening time constant (s)"
      settings: PortSchema="{\"entries\":[{\"content\":{\"sides\":[{\"content\":{\"connectorIds\":[\"LConn1\"]},\"type\":\"ConnectorPlacement.EquallySpacedRectSide\",\"uuid\":\"955749ca-45ab-4941-92ab-355bdf9f0774\"},{\"content\":{\"connectorIds\":[],\"side\":\"RIGHT\"},\"type\":\"ConnectorPlacement.EquallySpacedRectSide\",\"uuid\":\"c92dcc5f-a0c1-47cb-824d-a6fc82e3fc14\"},{\"content\":{\"connectorIds\":[\"LConn2\"],\"side\":\"TOP\"},\"type\":\"ConnectorPlacement.EquallySpacedRectSide\",\"uuid\":\"48cd19fd-8f40-4cf9-b8e1-bdcb1fb872a4\"},{\"content\":{\"connectorIds\":[\"RConn1\"],\"side\":\"BOTTOM\"},\"type\":\"ConnectorPlacement.EquallySpacedRectSide\",\"uuid\":\"979e7f94-a937-4bda-a98e-05d55fe22e7f\"},{\"content\":{\"connectorIds\":[],\"side\":\"HIDDEN\"},\"type\":\"ConnectorPlacement.EquallySpacedRectSide\",\"uuid\":\"a76ff1f3-0ae3-4e2b-93e3-18e3466b7d92\"}]},\"type\":\"ConnectorPlacement.EquallySpacedConnector\",\"uuid\":\"fbef87af-e9e5-4d13-8a42-ca228c07fa4c\"}],\"packageUris\":[\"http://schema.mathworks.com/mf0/Connector/R2020b\"],\"version\":\"1.0\"}"
  Scope{,1..6} (7 alike) : Scope
  Simulink-PS Converter : nesl_utility/Simulink-PS Converter  PhysicalDomain=network_engine_domain  SubClassName=ps_input  LeftPortType=input  RightPortType=output  PseudoPeriodic=off  Frequencies=[]  NoiseDistribution=none  NoiseParameters=[]  Unit=m^3/s  AffineConversion=off  FilteringAndDerivatives=provide  SimscapeFilterOrder=1  InputFilterTimeConstant=0.001  UdotUserProvided=0
  Simulink-PS Converter1 : nesl_utility/Simulink-PS Converter  PhysicalDomain=network_engine_domain  SubClassName=ps_input  LeftPortType=input  RightPortType=output  PseudoPeriodic=off  Frequencies=[]  NoiseDistribution=none  NoiseParameters=[]  Unit=degC  AffineConversion=on  FilteringAndDerivatives=provide  SimscapeFilterOrder=1  InputFilterTimeConstant=0.001  UdotUserProvided=0
  Simulink-PS Converter2 : nesl_utility/Simulink-PS Converter  PhysicalDomain=network_engine_domain  SubClassName=ps_input  LeftPortType=input  RightPortType=output  PseudoPeriodic=off  Frequencies=[]  NoiseDistribution=none  NoiseParameters=[]  Unit=MPa  AffineConversion=off  FilteringAndDerivatives=provide  SimscapeFilterOrder=1  InputFilterTimeConstant=0.001  UdotUserProvided=0
  Simulink-PS Converter3 : nesl_utility/Simulink-PS Converter  PhysicalDomain=network_engine_domain  SubClassName=ps_input  LeftPortType=input  RightPortType=output  PseudoPeriodic=off  Frequencies=[]  NoiseDistribution=none  NoiseParameters=[]  Unit=1  AffineConversion=off  FilteringAndDerivatives=provide  SimscapeFilterOrder=1  InputFilterTimeConstant=0.001  UdotUserProvided=0
  Simulink-PS Converter4 : nesl_utility/Simulink-PS Converter  PhysicalDomain=network_engine_domain  SubClassName=ps_input  LeftPortType=input  RightPortType=output  PseudoPeriodic=off  Frequencies=[]  NoiseDistribution=none  NoiseParameters=[]  Unit=1  AffineConversion=off  FilteringAndDerivatives=provide  SimscapeFilterOrder=1  InputFilterTimeConstant=0.001  UdotUserProvided=0
  Switch : Switch  Criteria=u2 > Threshold  SaturateOnIntegerOverflow=off  InputSameDT=off
  Transfer Fcn : TransferFcn  Denominator=[5 1]
  Transfer Fcn1 : TransferFcn  Denominator=[5 1]
  B : PMIOPort  Side=Left
  A : PMIOPort  Port=2  Side=Right
  tag scope: mfBlower=global
  wires:
  [T_env] -> Simulink-PS Converter1/1
  [p_env] -> Simulink-PS Converter2/1
  [CO2_env] -> Simulink-PS Converter4/1
  [cmd_blower] -> Scope1/1, Transfer Fcn/1
  [RH_env] -> Simulink-PS Converter3/1
  Transfer Fcn/1 -> Scope2/1, Max Flow [m^3/s]/1
  PS-Simulink Converter/1 -> Scope3/1
  PS-Simulink Converter1/1 -> Scope4/1
  [MPCController] -> Switch/2
  Max Flow [m^3/s]/1 -> Switch/3
  Switch/1 -> Scope/1, Scope5/1, [mfBlower], Simulink-PS Converter/1
  [cabAirMfIn] -> Transfer Fcn1/1
  Transfer Fcn1/1 -> Switch/1
  connections:
  Recirculation Flap/LConn2 -- Moist Air Properties/RConn1 -- Blower/LConn1
  Blower/RConn1 -- Flow Rate Sensor (MA)/LConn1 -- B/RConn1
  Environment Air/LConn1 -- Recirculation Flap/LConn1
  Simulink-PS Converter3/RConn1 -- Environment Air/RConn3
  Simulink-PS Converter1/RConn1 -- Environment Air/RConn1
  Blower/LConn2 -- Simulink-PS Converter/RConn1
  Recirculation Flap/RConn1 -- A/RConn1
  Simulink-PS Converter2/RConn1 -- Environment Air/RConn2
  Simulink-PS Converter4/RConn1 -- Environment Air/RConn4
  PS-Simulink Converter/LConn1 -- Flow Rate Sensor (MA)/RConn2
  PS-Simulink Converter1/LConn1 -- Flow Rate Sensor (MA)/RConn3
